simulink library "cntrlAltIndi_lib"  (R2018b)
settings: Solver=VariableStepAuto  StartTime=0.0  StopTime=10.0  RelTol=1e-3
undefined symbols (not defined in the file): DiscIntNeverNeededParam, psc
libraries: ndi_lib x1
settings Model: Creator=Ybeyer  LastModifiedBy=yannic
settings SFSimCC: SimUseLocalCustomCode=off
settings RTWCC: RTWUseLocalCustomCode=off
settings CodeAppCC: StateflowObjectComments=on

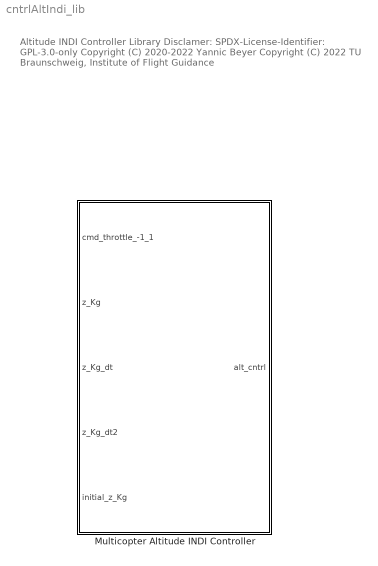
== system cntrlAltIndi_lib ==
  note: Altitude INDI Controller Library
      |
      | Disclamer:
      | SPDX-License-Identifier: GPL-3.0-only
      |
      | Copyright (C) 2020-2022 Yannic Beyer
      | Copyright (C) 2022 TU Braunschweig, Institute of Flight Guidance
  Multicopter Altitude INDI Controller : Subsystem  mask{psc=psc}
      mask prompts: psc "position control struct"
      mask DialogControl DescGroupVar Prompt: INDI Altitude Controller
      mask DialogControl DescTextVar Prompt: To initialize the position control struct see cntrlPosNdiLoadParams.

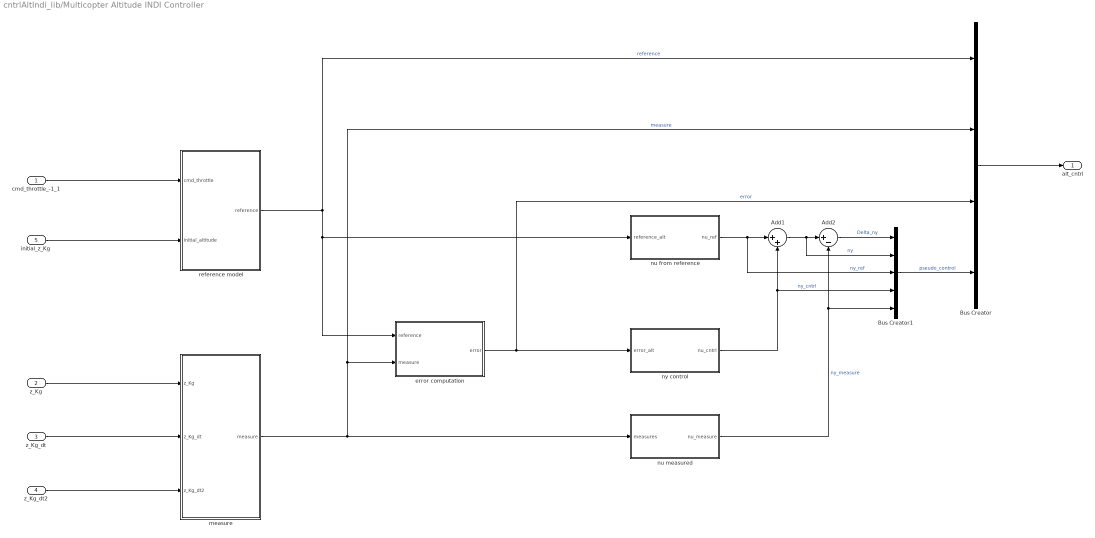
== system cntrlAltIndi_lib/Multicopter Altitude INDI Controller ==
  cmd_throttle_-1_1 : Inport
  z_Kg : Inport  Port=2
  z_Kg_dt : Inport  Port=3
  z_Kg_dt2 : Inport  Port=4
  initial_z_Kg : Inport  Port=5
  Add1 : Sum  Inputs=|++
  Add2 : Sum  Inputs=|+-
  Bus Creator : BusCreator  Inputs=4
  Bus Creator1 : BusCreator  Inputs=5
  error computation : Subsystem
  measure : Subsystem
  nu from reference : Subsystem
  nu measured : Subsystem
  ny control : Subsystem
  reference model : Subsystem
  alt_cntrl : Outport
  wires:
  nu from reference/1(nu_ref) -> Add1/1, Bus Creator1/3  "ny_ref"
  error computation/1(error) -> Bus Creator/3, ny control/1(error_alt)  "error"
  ny control/1(nu_cntrl) -> Add1/2, Bus Creator1/4  "ny_cntrl"
  nu measured/1(nu_measure) -> Add2/2, Bus Creator1/5  "ny_measure"
  reference model/1(reference) -> error computation/1(reference), nu from reference/1(reference_alt), Bus Creator/1  "reference"
  initial_z_Kg/1 -> reference model/2(initial_altitude)
  Bus Creator/1 -> alt_cntrl/1
  Bus Creator1/1 -> Bus Creator/4  "pseudo_control"
  Add2/1 -> Bus Creator1/1  "Delta_ny"
  measure/1(measure) -> nu measured/1(measures), Bus Creator/2, error computation/2(measure)  "measure"
  z_Kg_dt2/1 -> measure/3(z_Kg_dt2)
  z_Kg_dt/1 -> measure/2(z_Kg_dt)
  z_Kg/1 -> measure/1(z_Kg)
  cmd_throttle_-1_1/1 -> reference model/1(cmd_throttle)
  Add1/1 -> Bus Creator1/2, Add2/1  "ny"

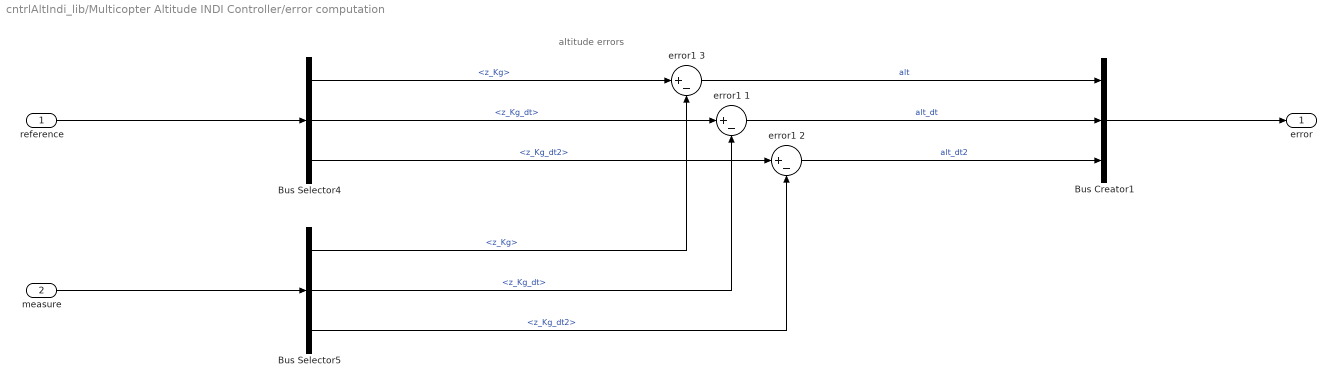
== system cntrlAltIndi_lib/Multicopter Altitude INDI Controller/error computation ==
  note: altitude errors
  reference : Inport
  measure : Inport  Port=2
  Bus Creator1 : BusCreator  Inputs=3
  Bus Selector4 : BusSelector  OutputSignals=z_Kg,z_Kg_dt,z_Kg_dt2
  Bus Selector5 : BusSelector  OutputSignals=z_Kg,z_Kg_dt,z_Kg_dt2
  error1 1 : Sum  Inputs=|+-
  error1 2 : Sum  Inputs=|+-
  error1 3 : Sum  Inputs=|+-
  error : Outport
  wires:
  Bus Selector4/2 -> error1 1/1  "<z_Kg_dt>"
  Bus Selector5/2 -> error1 1/2  "<z_Kg_dt>"
  reference/1 -> Bus Selector4/1
  measure/1 -> Bus Selector5/1
  Bus Selector4/3 -> error1 2/1  "<z_Kg_dt2>"
  Bus Selector5/3 -> error1 2/2  "<z_Kg_dt2>"
  Bus Selector4/1 -> error1 3/1  "<z_Kg>"
  Bus Selector5/1 -> error1 3/2  "<z_Kg>"
  error1 3/1 -> Bus Creator1/1  "alt"
  error1 1/1 -> Bus Creator1/2  "alt_dt"
  error1 2/1 -> Bus Creator1/3  "alt_dt2"
  Bus Creator1/1 -> error/1

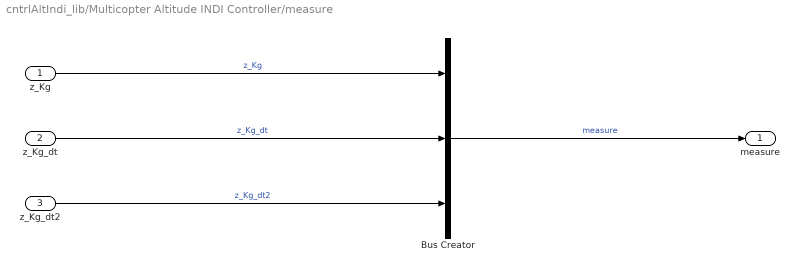
== system cntrlAltIndi_lib/Multicopter Altitude INDI Controller/measure ==
  z_Kg : Inport
  z_Kg_dt : Inport  Port=2
  z_Kg_dt2 : Inport  Port=3
  Bus Creator : BusCreator  Inputs=3
  measure : Outport
  wires:
  z_Kg/1 -> Bus Creator/1  "z_Kg"
  z_Kg_dt/1 -> Bus Creator/2  "z_Kg_dt"
  z_Kg_dt2/1 -> Bus Creator/3  "z_Kg_dt2"
  Bus Creator/1 -> measure/1  "measure"

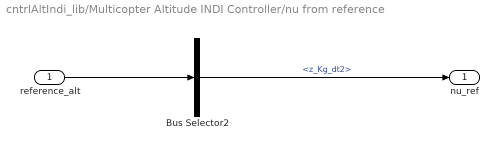
== system cntrlAltIndi_lib/Multicopter Altitude INDI Controller/nu from reference ==
  reference_alt : Inport
  Bus Selector2 : BusSelector  OutputSignals=z_Kg_dt2
  nu_ref : Outport
  wires:
  reference_alt/1 -> Bus Selector2/1
  Bus Selector2/1 -> nu_ref/1  "<z_Kg_dt2>"

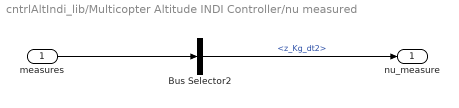
== system cntrlAltIndi_lib/Multicopter Altitude INDI Controller/nu measured ==
  measures : Inport
  Bus Selector2 : BusSelector  OutputSignals=altitude.z_Kg_dt2
  nu_measure : Outport
  wires:
  Bus Selector2/1 -> nu_measure/1  "<z_Kg_dt2>"
  measures/1 -> Bus Selector2/1

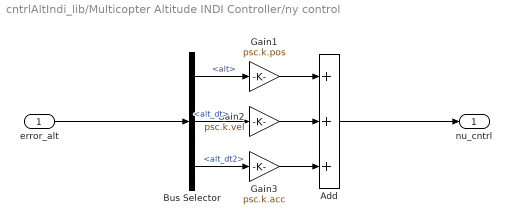
== system cntrlAltIndi_lib/Multicopter Altitude INDI Controller/ny control ==
  error_alt : Inport
  Add : Sum  Inputs=3
  Bus Selector : BusSelector  OutputSignals=alt,alt_dt,alt_dt2
  Gain1 : Gain  Gain=psc.k.pos
  Gain2 : Gain  Gain=psc.k.vel
  Gain3 : Gain  Gain=psc.k.acc
  nu_cntrl : Outport
  wires:
  error_alt/1 -> Bus Selector/1
  Add/1 -> nu_cntrl/1
  Bus Selector/1 -> Gain1/1  "<alt>"
  Bus Selector/2 -> Gain2/1  "<alt_dt>"
  Bus Selector/3 -> Gain3/1  "<alt_dt2>"
  Gain1/1 -> Add/1
  Gain2/1 -> Add/2
  Gain3/1 -> Add/3

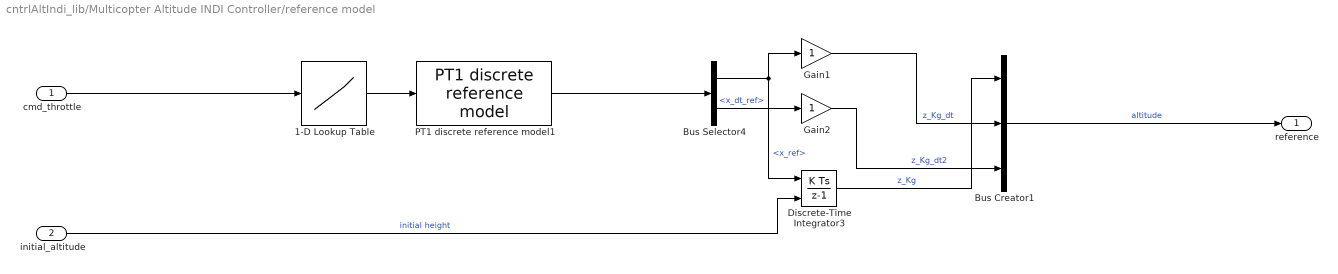
== system cntrlAltIndi_lib/Multicopter Altitude INDI Controller/reference model ==
  cmd_throttle : Inport
  initial_altitude : Inport  Port=2
  1-D Lookup Table : Lookup_n-D  NumberOfTableDimensions=1  BreakpointsForDimension1=[-1,0,1]  Table=[psc.rm.veldmax,0,-psc.rm.velumax]  InternalRulePriority=Speed  RndMeth=Simplest  InputSameDT=on
  Bus Creator1 : BusCreator  Inputs=3
  Bus Selector4 : BusSelector  OutputSignals=x_ref,x_dt_ref
  Discrete-Time Integrator3 : DiscreteIntegrator  InitialConditionSource=external  SampleTime=-1  ICPrevOutput=DiscIntNeverNeededParam  ICPrevScaledInput=DiscIntNeverNeededParam
  Gain1 : Gain
  Gain2 : Gain
  PT1 discrete reference model1 : ndi_lib/PT1 discrete reference model  T=psc.rm.veltc  x_max=inf  x_min=-inf  x_dt_max=psc.rm.accdmax  x_dt_min=-psc.rm.accumax  x_init=0
      settings: SourceProductName=LADAC
  reference : Outport
  wires:
  1-D Lookup Table/1 -> PT1 discrete reference model1/1
  cmd_throttle/1 -> 1-D Lookup Table/1
  Bus Selector4/1 -> Discrete-Time Integrator3/1, Gain1/1  "<x_ref>"
  PT1 discrete reference model1/1 -> Bus Selector4/1
  Bus Selector4/2 -> Gain2/1  "<x_dt_ref>"
  Bus Creator1/1 -> reference/1  "altitude"
  Discrete-Time Integrator3/1 -> Bus Creator1/1  "z_Kg"
  Gain1/1 -> Bus Creator1/2  "z_Kg_dt"
  Gain2/1 -> Bus Creator1/3  "z_Kg_dt2"
  initial_altitude/1 -> Discrete-Time Integrator3/2  "initial height"
